simulink model "microgrid_v1"  (R2025b)
settings: Solver=FixedStepDiscrete  StartTime=0.0  StopTime=86340  FixedStep=dt  RelTol=1e-3
undefined symbols (not defined in the file): DiscIntNeverNeededParam, dt, par_vec, SOC0
settings Model: Creator=Memad  LastModifiedBy=Memad

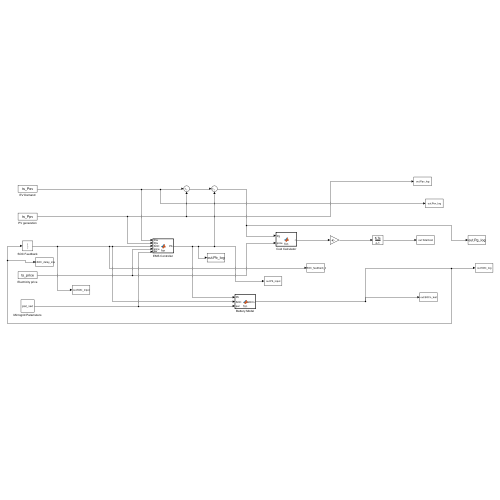
[thumbnail: Simulink's stored preview of the top-level diagram]
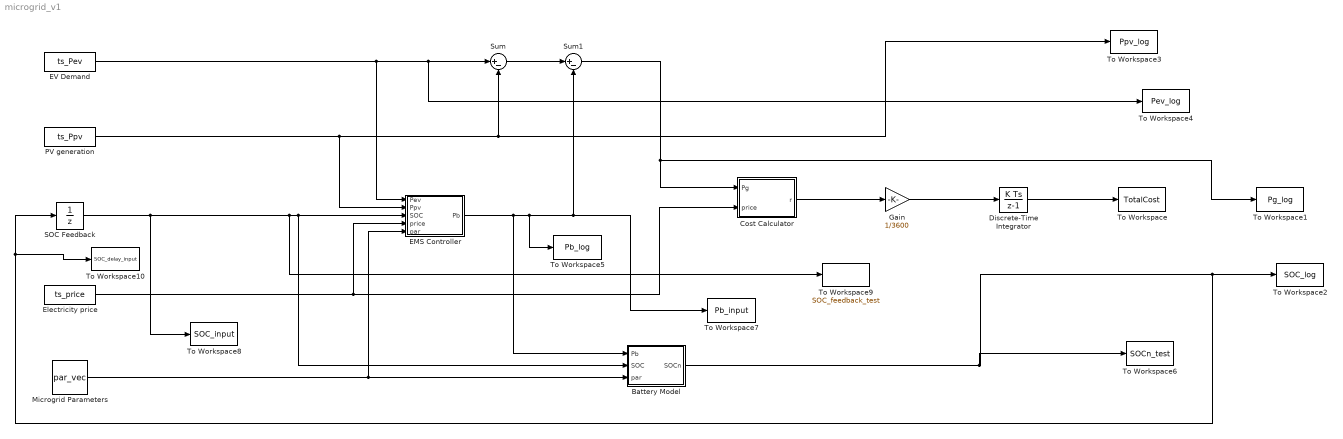
== system microgrid_v1 ==
  Battery Model : MATLAB Function  TreatAsAtomicUnit=on
  Cost Calculator : MATLAB Function  TreatAsAtomicUnit=on
  Discrete-Time Integrator : DiscreteIntegrator  SampleTime=dt  ICPrevOutput=DiscIntNeverNeededParam  ICPrevScaledInput=DiscIntNeverNeededParam
  EMS Controller : MATLAB Function  TreatAsAtomicUnit=on
  EV Demand : FromWorkspace  VariableName=ts_Pev  SampleTime=dt  Interpolate=off  OutputAfterFinalValue=Setting to zero
  Electricity price : FromWorkspace  VariableName=ts_price  SampleTime=dt  Interpolate=off  OutputAfterFinalValue=Setting to zero
  Gain : Gain  Gain=1/3600
  Microgrid Parameters : Constant  Value=par_vec
  PV generation : FromWorkspace  VariableName=ts_Ppv  SampleTime=dt  Interpolate=off  OutputAfterFinalValue=Setting to zero
  SOC Feedback : UnitDelay  InitialCondition=SOC0  SampleTime=dt  HasFrameUpgradeWarning=on
  Sum : Sum  Inputs=|+-
  Sum1 : Sum  Inputs=|+-
  To Workspace : ToWorkspace  VariableName=TotalCost  SaveFormat=Timeseries  SampleTime=-1
  To Workspace1 : ToWorkspace  VariableName=Pg_log  SaveFormat=Timeseries  SampleTime=-1
  To Workspace10 : ToWorkspace  VariableName=SOC_delay_input  SaveFormat=Timeseries  SampleTime=-1
  To Workspace2 : ToWorkspace  VariableName=SOC_log  SaveFormat=Timeseries  SampleTime=-1
  To Workspace3 : ToWorkspace  VariableName=Ppv_log  SaveFormat=Timeseries  SampleTime=-1
  To Workspace4 : ToWorkspace  VariableName=Pev_log  SaveFormat=Timeseries  SampleTime=-1
  To Workspace5 : ToWorkspace  VariableName=Pb_log  SaveFormat=Timeseries  SampleTime=-1
  To Workspace6 : ToWorkspace  VariableName=SOCn_test  SaveFormat=Timeseries  SampleTime=-1
  To Workspace7 : ToWorkspace  VariableName=Pb_input  SaveFormat=Timeseries  SampleTime=-1
  To Workspace8 : ToWorkspace  VariableName=SOC_input  SaveFormat=Timeseries  SampleTime=-1
  To Workspace9 : ToWorkspace  VariableName=SOC_feedback_test  SaveFormat=Timeseries  SampleTime=-1
  wires:
  EV Demand/1 -> To Workspace4/1, Sum/1, EMS Controller/1(Pev)
  PV generation/1 -> To Workspace3/1, Sum/2, EMS Controller/2(Ppv)
  SOC Feedback/1 -> To Workspace8/1, To Workspace9/1, EMS Controller/3(SOC), Battery Model/2(SOC)
  Electricity price/1 -> EMS Controller/4(price), Cost Calculator/2(price)
  Microgrid Parameters/1 -> EMS Controller/5(par), Battery Model/3(par)
  EMS Controller/1(Pb) -> To Workspace5/1, To Workspace7/1, Sum1/2, Battery Model/1(Pb)
  Sum/1 -> Sum1/1
  Sum1/1 -> To Workspace1/1, Cost Calculator/1(Pg)
  Gain/1 -> Discrete-Time Integrator/1
  Cost Calculator/1(r) -> Gain/1
  Discrete-Time Integrator/1 -> To Workspace/1
  Battery Model/1(SOCn) -> To Workspace6/1, To Workspace10/1, SOC Feedback/1, To Workspace2/1

== matlab function microgrid_v1/Battery Model ==
  data: Pb input; SOCn output; SOC input; par input
function SOCn = fcn(Pb, SOC, par)

SOCmin = par(2);
SOCmax = par(3);
Ebat = par(4);
eta = par(8);
dt = par(9);

if Pb >= 0
    % Discharging
    dE = -Pb / eta * dt / 3600;
else
    % Charging
    dE = -Pb * eta * dt / 3600;
end

SOCn = SOC + dE / Ebat;

SOCn = min(max(SOCn, SOCmin), SOCmax);

end

== matlab function microgrid_v1/EMS Controller ==
  data: Pev input; Pb output; Ppv input; SOC input; price input; par input
function Pb = fcn(Pev, Ppv, SOC, price, par)

% Extract parameters
Pbmax = par(1);
SOCmin = par(2);
SOCmax = par(3);
Ebat = par(4);
Pgrid_target = par(5);
price_hi = par(6);
price_lo = par(7);
eta = par(8);
dt = par(9);
Gmax = par(10);

% Calculate net power
Net = Pev - Ppv;

% Default battery power
Pb = 0;

% Energy management strategy
if Net < 0
    Pb = max(Net, -Pbmax);

elseif price >= price_hi || Net > Pgrid_target
    Pb = min(Net, Pbmax);

elseif price <= price_lo && SOC < 0.5
    Pb = -0.5 * Pbmax;
end

% SOC constraints
Pdischarge_SOC = max(0, (SOC-SOCmin)*Ebat*eta*3600/dt);
Pcharge_SOC = max(0, (SOCmax-SOC)*Ebat*3600/(eta*dt));

Pb = min(Pb, Pdischarge_SOC);
Pb = max(Pb, -Pcharge_SOC);

% Battery power constraints
Pb = min(max(Pb,-Pbmax),Pbmax);

% Grid import constraint
if Net-Pb > Gmax
    Pb = max(Pb,Net-Gmax);
end

end

== matlab function microgrid_v1/Cost Calculator ==
  data: Pg input; r output; price input
function r = fcn(Pg, price)

feedin = 0.08;

r = max(Pg, 0)*price - max(-Pg, 0)*feedin;

end
